simulink model "SimulinkStateSpace"  (R2024b)
settings: Solver=ode45  StartTime=0.0  StopTime=tEnd  MaxStep=1  RelTol=1e-6
values from neighbouring files (symbols this model uses):
  A = [0       0    1     0 ... (first row only)    [FinalSettingsForObserverControl.m]    (also in StateSpaceInitialization.m)
  B = [0       0 ... (first row only)    [FinalSettingsForObserverControl.m]    (also in StateSpaceInitialization.m)
  C = eye(4)    [StateSpaceInitialization.m]
  D = zeros(4,2)    [StateSpaceInitialization.m]
  K = [kp + 3*mc*n^2,  0,    kd,       2*mc*n ... (first row only)    [FinalSettingsForObserverControl.m]    (also in StateSpaceInitialization.m = place(A,B,poles))
  z0 = [x0; y0; vx0; vy0]    [FinalSettingsForObserverControl.m]    (also in StateSpaceInitialization.m = [10; 0; 0; 0])
settings Model: Creator=USER  LastModifiedBy=USER

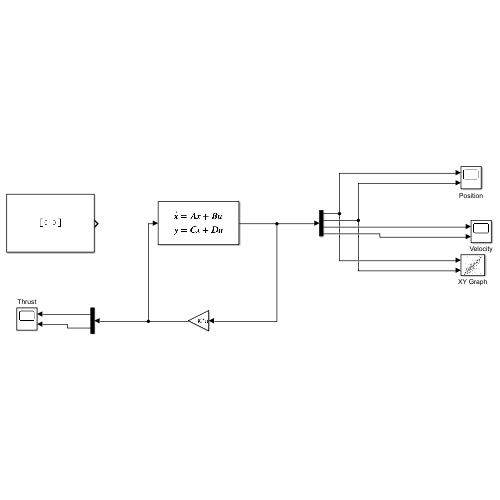
[thumbnail: Simulink's stored preview of the top-level diagram]
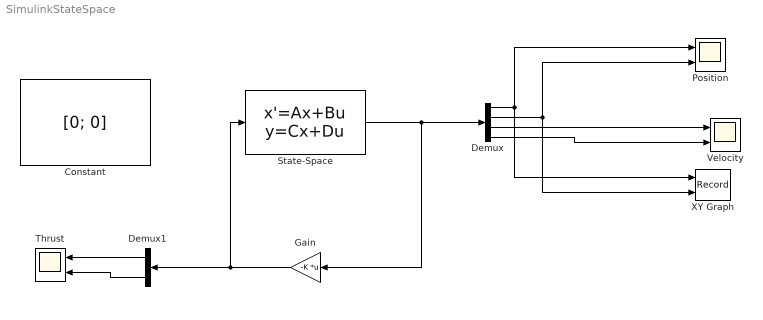
== system SimulinkStateSpace ==
  Constant : Constant  Value=[0; 0]
  Demux : Demux
  Demux1 : Demux  Outputs=2
  Gain : Gain  Gain=-K  Multiplication=Matrix(K*u)
  Position : Scope  NumInputPorts=2
  State-Space : StateSpace  A=A  B=B  C=C  D=D  InitialCondition=z0
  Thrust : Scope  NumInputPorts=2
  Velocity : Scope  NumInputPorts=2
  XY Graph : Record  FileSettingsInternal="{\"entries\":[{\"content\":{\"excelSettings\":{\"content\":{},\"type\":\"Streamout.ExcelSettings\"}},\"type\":\"Streamout.FileSettingStorage\",\"uuid\":\"\"}],\"packageUris\":[\"http:\\/\\/schema.mathworks.com\\/mf0\\/streamout_blocks\\/R2020a\"],\"version\":\"1.0\"}"  Layout=[1 1]  SignalsInternal="{\"entries\":[{\"content\":{\"signals\":[{\"content\":{\"blockPath\":[],\"dimensions\":[1],\"domain\":\"\",\"lineColor\":\"#a2142f\",\"plots\":[ 1 ],\"port\":1,\"sid\":[\"\"],\"signalID\":1,\"signalName\":\"Demux:1\"},\"type\":\"RecordBlkView.Signal\",\"uuid\":\"\"},{\"content\":{\"blockPath\":[],\"dimensions\":[1],\"domain\":\"\",\"lineColor\":\"#139fff\",\"plots\":[ 1 ],\"port\":2,\"sid\":[\"\"],\"signalID\":2,\"signalName\":\"Demux:2\"},\"type\":\"RecordBlkView.Signal\",\"uuid\":\"\"}]},\"type\":\"RecordBlkView.InputSignals\",\"uuid\":\"\"}],\"packageUris\":[\"http:\\/\\/schema.mathworks.com\\/mf0\\/streamout_blocks\\/R2020a\"],\"version\":\"1.0\"}"  VisualizationBindings="{\"xyplotplugin\":{\"info\":[{\"series\":[{\"bindingParametersList\":[{\"parameter\":\"X-Axis\",\"signalID\":1,\"signalName\":\"Demux:1\"},{\"parameter\":\"Y-Axis\",\"signalID\":2,\"signalName\":\"Demux:2\"}],\"seriesID\":0}],\"subplotID\":1}]}}"  CompatibilityTag=XY
  wires:
  State-Space/1 -> Gain/1, Demux/1
  Demux/1 -> XY Graph/1, Position/1
  Demux/2 -> XY Graph/2, Position/2
  Demux/3 -> Velocity/1
  Demux/4 -> Velocity/2
  Gain/1 -> Demux1/1, State-Space/1
  Demux1/1 -> Thrust/1
  Demux1/2 -> Thrust/2
